simulink model "My_gfm_battery_sil_2_ConvIGBT_zDomain"  (R2025b)
settings: Solver=ode23t  StartTime=0.0  StopTime=10  MaxStep=1e-4  RelTol=1e-3
PreLoadFcn:
  | close all;
  | clear all;
  | clc;
  | 
  | 
  | modelDir = fileparts(get_param(bdroot,'FileName'));
  | 
  | load_system(fullfile(modelDir,'controls_element_lib.slx'));
  | load_system(fullfile(modelDir,'test_sequence_lib.slx'));
  | 
  | Simulink.importExternalCTypes('.\circuitControls_A_autogen.h')
InitFcn:
  | % frequency nominals
  | F_NOM = 60;
  | W_NOM = 2 * pi * F_NOM;
  | 
  | % base values relative to inverter
  | % --------------------------------
  | VLL_INV_NOM = 480;
  | P_INV_NOM = 1e6;
  | Q_INV_NOM = 0.5e6;
  | S_INV_NOM = sqrt(P_INV_NOM^2 + Q_INV_NOM^2);
  | 
  | I_INV_BASE = S_INV_NOM/(sqrt(3)*VLL_INV_NOM);
  | Z_INV_BASE = VLL_INV_NOM^2/S_INV_NOM;
  | L_INV_BASE = Z_INV_BASE / W_NOM;
  | C_INV_BASE = 1 / (Z_INV_BASE * W_NOM);
  | 
  | % nominal ratings for power system model
  | % --------------------------------------
  | INVERTER_COUNT = 100;
  | 
  | VLV_NOM = VLL_INV_NOM;
  | VMV_NOM = 35e3;
  | VHV_NOM = 230e3;
  | S_PLANT = INVERTER_COUNT * S_INV_NOM;
  | 
  | N_GSU = VHV_NOM/VMV_NOM;
  | N_MVT = VMV_NOM/VLV_NOM;
  | 
  | I_LV_BASE = S_PLANT/(sqrt(3)*VLV_NOM);
  | I_MV_BASE = S_PLANT/(sqrt(3)*VMV_NOM);
  | I_HV_BASE = S_PLANT/(sqrt(3)*VHV_NOM);
  | 
  | Z_LV_BASE = VLV_NOM^2/S_PLANT;
  | Z_MV_BASE = VMV_NOM^2/S_PLANT;
  | Z_HV_BASE = VHV_NOM^2/S_PLANT;
  | 
  | L_LV_BASE = Z_LV_BASE / W_NOM;
  | L_MV_BASE = Z_MV_BASE / W_NOM;
  | L_HV_BASE = Z_HV_BASE / W_NOM;
  | C_LV_BASE = 1 / (Z_LV_BASE * W_NOM);
  | C_MV_BASE = 1 / (Z_MV_BASE * W_NOM);
  | C_HV_BASE = 1 / (Z_HV_BASE * W_NOM);
undefined symbols (not defined in the file): D1, D11, Delta, gcbh, j, powergui, SampleTime, sps_rtmsupport, Ts
libraries: simulink x43, spsVoltageMeasurementLib x21, spsThreePhaseSeriesRLCBranchLib x20, spsControlledCurrentSourceLib x20, spsControlledVoltageSourceLib x15, spsThreePhaseVIMeasurementLib x12, spsSeriesRLCBranchLib x11, spsGroundLib x11, test_sequence_lib x10, controls_element_lib x9, spsCurrentMeasurementLib x8, spsThreePhaseTransformerTwoWindingsLib x6
(part 7 of 8)

== system My_gfm_battery_sil_2_ConvIGBT_zDomain/My Inverter Controller /My_machineModel_A/Exciter ==
  note: Aligning with Rotor Frame
      | cos x + j sin x
      | cos (x-120) + j (sin x -120)
      | cos (x+120) + j (sin x +120)
  note: Vb = vd * cos (x-120) - vq * sin (x-120)
  note: Peak EMFa,b,c
  note: Va = vd * cos x - vq * sin x
  note: Vq = 0
  note: Vc = vd * cos (x+120) - vq * sin (x+120)
  Vexc : Inport
  osc[3] : Inport  Port=2
  Constant : Constant  Value=0
  Gain2 : Gain  Gain=1/sqrt(3)
  LPF : Subsystem
  LPF1 : TransferFcn  Commented=on  Denominator=[1/wExciter 1]
  Real-Imag to Complex : RealImagToComplex
  modulator : Subsystem
  v_emf : Outport
  wires:
  LPF/1(Out) -> Gain2/1  "Vref_LL"
  modulator/1(ref) -> v_emf/1
  Gain2/1 -> Real-Imag to Complex/1  "Vref_LN"
  osc[3]/1 -> modulator/2(osc)
  Constant/1 -> Real-Imag to Complex/2
  Real-Imag to Complex/1 -> modulator/1(cmd)
  Vexc/1 -> LPF/1(In)

== system My_gfm_battery_sil_2_ConvIGBT_zDomain/My Inverter Controller /My_machineModel_A/governer ==
  note: Machine enables
  note: RMS LL
  note: RMS LL
  note: Machine Disabled, Power sync on
  Prequest : Inport
  Fref : Inport  Port=2
  enabled : Inport  Port=3
  Vt : Inport  Port=4
  Vq : Inport  Port=5
  f_rotor : Inport  Port=6
  "LPF(DamperDecoupler) limited " : Subsystem
  Saturation1 : Saturate  UpperLimit=nominalFrequency+1  LowerLimit=nominalFrequency-1
  Scope1 : Scope  NumInputPorts=4
      settings: ActiveDisplayYMinimum=-3.88223850701E+6  ActiveDisplayYMaximum=1.39902720117E+6
  Scope2 : Scope  NumInputPorts=3
      settings: ActiveDisplayYMinimum=-4.19262745781E+6  ActiveDisplayYMaximum=4.19262745781E+6  DataLoggingVariableName=ScopeData2
  Sum : Sum  Inputs=|++
  Sum1 : Sum  Inputs=|+-
  Sum2 : Sum  Inputs=++|
  droop power limits : Saturate  UpperLimit=SRated  LowerLimit=-SRated
  k_droop : Gain  Gain=kDroop * SRated
  power request limits : Saturate  UpperLimit=SRated  LowerLimit=-SRated
  synchronizer : Subsystem
  power : Outport
  wires:
  power request limits/1 -> Scope1/1, Sum2/1
  droop power limits/1 -> Sum2/2
  synchronizer/1(p_sync_pu) -> Scope2/1, Sum/2  "p_sync"
  Vq/1 -> synchronizer/1(Vq), Scope2/2
  Prequest/1 -> power request limits/1
  k_droop/1 -> droop power limits/1
  Sum2/1 -> Scope1/2, "LPF(DamperDecoupler) limited "/1(In)
  "LPF(DamperDecoupler) limited "/1(Out) -> Scope1/3, Sum/1  "p_mechanical"
  Saturation1/1 -> Sum1/1
  f_rotor/1 -> Sum1/2
  Fref/1 -> Saturation1/1
  Sum/1 -> Scope1/4, power/1
  Sum1/1 -> k_droop/1
  Vt/1 -> synchronizer/2(Vt), Scope2/3
  enabled/1 -> synchronizer/3(machine_enabled)

== system My_gfm_battery_sil_2_ConvIGBT_zDomain/My Inverter Controller /My_machineModel_A/impedance emulation ==
  v_emf : Inport
  enable : Inport  Port=2
  v_terminal : Inport  Port=3
  Constant : Constant  Value=0
  Integrator : Integrator
  Sum : Sum  Inputs=|+-
  Sum of Elements1 : Sum  Inputs=+
  Sum1 : Sum  Inputs=|+-
  Sum4 : Sum  Inputs=|+-
  Switch : Switch  Criteria=u2 > Threshold  SaturateOnIntegerOverflow=off  InputSameDT=off
  overLs : Gain  Gain=2*pi*60/(Xs * (VllRated^2/SRated))
  rN : Gain  Gain=rn*(VllRated^2/SRated)
  rs : Gain  Gain=rs*(VllRated^2/SRated)
  i_ref : Outport
  wires:
  enable/1 -> Switch/2
  Constant/1 -> Switch/3
  Sum/1 -> Switch/1
  Switch/1 -> Sum4/1
  v_terminal/1 -> Sum/2
  v_emf/1 -> Sum/1
  overLs/1 -> Integrator/1
  Sum of Elements1/1 -> rN/1
  Sum4/1 -> Sum1/1
  Sum1/1 -> overLs/1
  rN/1 -> Sum4/2
  rs/1 -> Sum1/2
  Integrator/1 -> Sum of Elements1/1, rs/1, i_ref/1  "i_ref"

== system My_gfm_battery_sil_2_ConvIGBT_zDomain/My Inverter Controller /My_machineModel_A/power analyzer ==
  iac : Inport
  vac : Inport  Port=2
  Demux1 : Demux  Outputs=3
  Demux2 : Demux  Outputs=3
  Gain3 : Gain  Gain=1 / sqrt(3)
  Product{,1..3} (4 alike) : Product
  Sum of Elements : Sum  Inputs=+
  Sum2 : Sum  Inputs=|+-
  Sum3 : Sum  Inputs=|+-
  Sum4 : Sum  Inputs=|+-
  Sum5 : Sum  Inputs=+++
  P : Outport
  Q : Outport  Port=2
  wires:
  Product/1 -> Sum of Elements/1
  Sum of Elements/1 -> P/1  "P"
  Gain3/1 -> Q/1  "Q"
  Demux1/1 -> Product2/2  "ia"
  Demux2/1 -> Sum2/1, Sum4/2
  Sum2/1 -> Product1/1  "vab"
  Sum5/1 -> Gain3/1
  Sum3/1 -> Product2/1  "vbc"
  iac/1 -> Demux1/1, Product/1
  vac/1 -> Product/2, Demux2/1
  Demux1/2 -> Product3/2  "ib"
  Demux1/3 -> Product1/2  "ic"
  Demux2/3 -> Sum3/2, Sum4/1
  Demux2/2 -> Sum2/2, Sum3/1
  Product3/1 -> Sum5/2
  Sum4/1 -> Product3/1  "vca"
  Product2/1 -> Sum5/3
  Product1/1 -> Sum5/1

== system My_gfm_battery_sil_2_ConvIGBT_zDomain/My Inverter Controller /My_machineModel_A/rotor model ==
  p_mechanical : Inport
  p_electrical : Inport  Port=2
  Constant : Constant  Value=nominalFrequency
  HPF (wDamperDecoupler) : TransferFcn  Commented=on  Numerator=[0.3 0]  Denominator=[0.3 1]
  HPF (wDamperDecoupler) 1 : Subsystem
  Integrator1 : Integrator  LimitOutput=on  UpperSaturationLimit=5  LowerSaturationLimit=-5
  Sum : Sum  Inputs=++|
  Sum2 : Sum  Inputs=|+-
  Sum3 : Sum  Inputs=|+-
  k_damp : Gain  Gain=kDamper*SRated
  k_inertia : Gain  Gain=(nominalFrequency/2)/(inertialConstant*SRated)
  oscillator_3ph : Subsystem
  osc[3] : Outport
  f_rotor : Outport  Port=2
  wires:
  Constant/1 -> Sum/1
  Sum/1 -> oscillator_3ph/1(f), f_rotor/1
  k_damp/1 -> Sum2/2
  Integrator1/1 -> HPF (wDamperDecoupler) 1/1(in), Sum/2
  p_mechanical/1 -> Sum3/1
  Sum3/1 -> Sum2/1
  p_electrical/1 -> Sum3/2
  HPF (wDamperDecoupler) 1/1(out) -> k_damp/1
  oscillator_3ph/1(osc[3]) -> osc[3]/1
  k_inertia/1 -> Integrator1/1
  Sum2/1 -> k_inertia/1

== system My_gfm_battery_sil_2_ConvIGBT_zDomain/My Inverter Controller /My_machineModel_A/voltage analyzer ==
  osc[3] : Inport
  v_terminal : Inport  Port=2
  Complex to Magnitude-Angle : ComplexToMagnitudeAngle
  Complex to Real-Imag : ComplexToRealImag
  Conj : Math  Operator=conj  SignedPower=on
  LPF : Subsystem
  "LPF " : Subsystem
  Product1 : Product
  Product2 : Product
  Real-Imag to Complex1 : RealImagToComplex
  Sum of Elements1 : Sum  Inputs=+
  Sum of Elements2 : Sum  Inputs=+
  Terminator : Terminator
  over_sqrt(3) : Gain  Gain=1/sqrt(3)
  over_sqrt(3)1 : Gain  Gain=1/sqrt(3)
  sqrt(2) : Gain  Gain=sqrt(2)
  Vd : Outport
  Vq : Outport  Port=2
  Vt_Mag : Outport  Port=3
  wires:
  "LPF "/1(Out) -> Real-Imag to Complex1/2, Vq/1  "Vq"
  osc[3]/1 -> Conj/1
  LPF/1(Out) -> Real-Imag to Complex1/1, Vd/1  "Vd"
  over_sqrt(3)1/1 -> LPF/1(In)
  over_sqrt(3)/1 -> "LPF "/1(In)
  Complex to Real-Imag/1 -> Product2/1
  Complex to Real-Imag/2 -> Product1/1
  Sum of Elements2/1 -> over_sqrt(3)1/1
  v_terminal/1 -> Product2/2, Product1/2
  Product1/1 -> Sum of Elements1/1
  Sum of Elements1/1 -> over_sqrt(3)/1
  sqrt(2)/1 -> Complex to Real-Imag/1
  Conj/1 -> sqrt(2)/1
  Product2/1 -> Sum of Elements2/1
  Complex to Magnitude-Angle/1 -> Vt_Mag/1  "Vt"
  Real-Imag to Complex1/1 -> Complex to Magnitude-Angle/1  "Vd"
  Complex to Magnitude-Angle/2 -> Terminator/1

== system My_gfm_battery_sil_2_ConvIGBT_zDomain/My Inverter Controller /My_machineModel_A1/excitation ==
  note: This limit is needed to avoid excessive currents during blackstart that cause windup in current limiting logic.. It results in a linear ramp of voltage during blackstart
  note: Using asym filter to traget long extended low voltage events, prevent it from acting during typical faults
  note: Aligning with Rotor Frame
      | cos x + j sin x
      | cos (x-120) + j (sin x -120)
      | cos (x+120) + j (sin x +120)
  note: Vb = vd * cos (x-120) - vq * sin (x-120)
  note: Peak EMFa,b,c
  note: Va = vd * cos x - vq * sin x
  note: Vq = 0
  note: Vc = vd * cos (x+120) - vq * sin (x+120)
  VRef : Inport
  osc[3] : Inport  Port=2
  Vt : Inport  Port=3
  Constant : Constant  Value=0
  Gain2 : Gain  Gain=1/sqrt(3)
  LPF : Subsystem
  LPF1 : TransferFcn  Commented=on  Denominator=[1/wExciter 1]
  Min : MinMax  Inputs=2
  Real-Imag to Complex : RealImagToComplex
  Saturation1 : Saturate  UpperLimit=1.1*VllRated  LowerLimit=0.9*VllRated
  Sum : Sum  Inputs=++|
  assymmetric filter1 : Subsystem
  modulator : Subsystem
  voltage_headroom : Constant  Value=0.3*VllRated
  v_emf : Outport
  wires:
  Sum/1 -> Min/2
  Saturation1/1 -> Min/1
  voltage_headroom/1 -> Sum/1
  LPF/1(Out) -> Gain2/1  "Vref_LL"
  Min/1 -> LPF/1(In)
  VRef/1 -> Saturation1/1  "VRef"
  modulator/1(ref) -> v_emf/1
  assymmetric filter1/1(out) -> Sum/2  "Vt_conditioned"
  Vt/1 -> assymmetric filter1/1(in)  "Vt"
  Gain2/1 -> Real-Imag to Complex/1  "Vref_LN"
  osc[3]/1 -> modulator/2(osc)
  Constant/1 -> Real-Imag to Complex/2
  Real-Imag to Complex/1 -> modulator/1(cmd)

== system My_gfm_battery_sil_2_ConvIGBT_zDomain/My Inverter Controller /My_machineModel_A1/governer ==
  note: Machine enables
  note: RMS LL
  note: RMS LL
  note: Machine Disabled, Power sync on
  Prequest : Inport
  Fref : Inport  Port=2
  enabled : Inport  Port=3
  Vt : Inport  Port=4
  Vq : Inport  Port=5
  f_rotor : Inport  Port=6
  "LPF(DamperDecoupler) limited " : Subsystem
  Saturation1 : Saturate  UpperLimit=nominalFrequency+1  LowerLimit=nominalFrequency-1
  Scope1 : Scope  NumInputPorts=4
      settings: ActiveDisplayYMinimum=-3.88223850701E+6  ActiveDisplayYMaximum=1.39902720117E+6
  Scope2 : Scope  NumInputPorts=3
      settings: ActiveDisplayYMinimum=-4.19262745781E+6  ActiveDisplayYMaximum=4.19262745781E+6  DataLoggingVariableName=ScopeData2
  Sum : Sum  Inputs=|++
  Sum1 : Sum  Inputs=|+-
  Sum2 : Sum  Inputs=++|
  droop power limits : Saturate  UpperLimit=SRated  LowerLimit=-SRated
  k_droop : Gain  Gain=kDroop * SRated
  power request limits : Saturate  UpperLimit=SRated  LowerLimit=-SRated
  synchronizer : Subsystem
  power : Outport
  wires:
  power request limits/1 -> Scope1/1, Sum2/1
  droop power limits/1 -> Sum2/2
  synchronizer/1(p_sync_pu) -> Scope2/1, Sum/2  "p_sync"
  Vq/1 -> Scope2/2, synchronizer/1(Vq)
  Prequest/1 -> power request limits/1
  k_droop/1 -> droop power limits/1
  Sum2/1 -> Scope1/2, "LPF(DamperDecoupler) limited "/1(In)
  "LPF(DamperDecoupler) limited "/1(Out) -> Scope1/3, Sum/1  "p_mechanical"
  Saturation1/1 -> Sum1/1
  f_rotor/1 -> Sum1/2
  Fref/1 -> Saturation1/1
  Sum/1 -> Scope1/4, power/1
  Sum1/1 -> k_droop/1
  Vt/1 -> Scope2/3, synchronizer/2(Vt)
  enabled/1 -> synchronizer/3(machine_enabled)

== system My_gfm_battery_sil_2_ConvIGBT_zDomain/My Inverter Controller /My_machineModel_A1/governer1 ==
  note: Machine enables
  note: RMS LL
  note: RMS LL
  note: Machine Disabled, Power sync on
  Prequest : Inport
  Fref : Inport  Port=2
  enabled : Inport  Port=3
  Vd : Inport  Port=4
  Vq : Inport  Port=5
  f_rotor : Inport  Port=6
  LPF(DamperDecoupler) - limited : Subsystem  Commented=on
  LPF(DamperDecoupler) limited 1 : Subsystem
  Saturation1 : Saturate  UpperLimit=nominalFrequency+1  LowerLimit=nominalFrequency-1
  Sum : Sum  Inputs=|++
  Sum1 : Sum  Inputs=|+-
  Sum2 : Sum  Inputs=++|
  droop power limits : Saturate  UpperLimit=SRated  LowerLimit=-SRated
  k_droop : Gain  Gain=kDroop * SRated
  power request limits : Saturate  UpperLimit=SRated  LowerLimit=-SRated
  synchronizer : Subsystem
  power : Outport
  wires:
  power request limits/1 -> Sum2/1
  droop power limits/1 -> Sum2/2
  synchronizer/1(p_sync_pu) -> Sum/2  "p_sync"
  Vq/1 -> synchronizer/1(Vq)
  Prequest/1 -> power request limits/1
  k_droop/1 -> droop power limits/1
  Sum2/1 -> LPF(DamperDecoupler) limited 1/1(In)
  enabled/1 -> synchronizer/3(machine_enabled)
  LPF(DamperDecoupler) limited 1/1(Out) -> Sum/1  "p_mechanical"
  Saturation1/1 -> Sum1/1
  f_rotor/1 -> Sum1/2
  Fref/1 -> Saturation1/1
  Sum/1 -> power/1
  Sum1/1 -> k_droop/1
  Vd/1 -> synchronizer/2(Vd)

== system My_gfm_battery_sil_2_ConvIGBT_zDomain/My Inverter Controller /My_machineModel_A1/impedance emulation ==
  v_emf : Inport
  enable : Inport  Port=2
  v_terminal : Inport  Port=3
  Constant : Constant  Value=0
  Integrator : Integrator
  Sum : Sum  Inputs=|+-
  Sum of Elements1 : Sum  Inputs=+
  Sum1 : Sum  Inputs=|+-
  Sum4 : Sum  Inputs=|+-
  Switch : Switch  Criteria=u2 > Threshold  SaturateOnIntegerOverflow=off  InputSameDT=off
  overLs : Gain  Gain=2*pi*60/(Xs * (VllRated^2/SRated))
  rN : Gain  Gain=0.2*(VllRated^2/SRated)
  rs : Gain  Gain=rs*(VllRated^2/SRated)
  i_ref : Outport
  wires:
  enable/1 -> Switch/2
  Constant/1 -> Switch/3
  Sum/1 -> Switch/1
  Switch/1 -> Sum4/1
  v_terminal/1 -> Sum/2
  v_emf/1 -> Sum/1
  overLs/1 -> Integrator/1
  Sum of Elements1/1 -> rN/1
  Sum4/1 -> Sum1/1
  Sum1/1 -> overLs/1
  rN/1 -> Sum4/2
  rs/1 -> Sum1/2
  Integrator/1 -> Sum of Elements1/1, rs/1, i_ref/1  "i_ref"

== system My_gfm_battery_sil_2_ConvIGBT_zDomain/My Inverter Controller /My_machineModel_A1/power analyzer ==
  iac : Inport
  vac : Inport  Port=2
  Demux1 : Demux  Outputs=3
  Demux2 : Demux  Outputs=3
  Gain3 : Gain  Gain=1 / sqrt(3)
  Product{,1..3} (4 alike) : Product
  Sum of Elements : Sum  Inputs=+
  Sum2 : Sum  Inputs=|+-
  Sum3 : Sum  Inputs=|+-
  Sum4 : Sum  Inputs=|+-
  Sum5 : Sum  Inputs=+++
  P : Outport
  Q : Outport  Port=2
  wires:
  Product/1 -> Sum of Elements/1
  Sum of Elements/1 -> P/1  "P"
  Gain3/1 -> Q/1  "Q"
  Demux1/1 -> Product2/2  "ia"
  Demux2/1 -> Sum2/1, Sum4/2
  Sum2/1 -> Product1/1  "vab"
  Sum5/1 -> Gain3/1
  Sum3/1 -> Product2/1  "vbc"
  iac/1 -> Demux1/1, Product/1
  vac/1 -> Product/2, Demux2/1
  Demux1/2 -> Product3/2  "ib"
  Demux1/3 -> Product1/2  "ic"
  Demux2/3 -> Sum3/2, Sum4/1
  Demux2/2 -> Sum2/2, Sum3/1
  Product3/1 -> Sum5/2
  Sum4/1 -> Product3/1  "vca"
  Product2/1 -> Sum5/3
  Product1/1 -> Sum5/1

== system My_gfm_battery_sil_2_ConvIGBT_zDomain/My Inverter Controller /My_machineModel_A1/rotor model ==
  p_mechanical : Inport
  p_electrical : Inport  Port=2
  Constant : Constant  Value=nominalFrequency
  HPF (wDamperDecoupler) : TransferFcn  Commented=on  Numerator=[0.3 0]  Denominator=[0.3 1]
  HPF (wDamperDecoupler) 1 : Subsystem
  Integrator1 : Integrator  LimitOutput=on  UpperSaturationLimit=5  LowerSaturationLimit=-5
  Sum : Sum  Inputs=++|
  Sum2 : Sum  Inputs=|+-
  Sum3 : Sum  Inputs=|+-
  k_damp : Gain  Gain=kDamper*SRated
  k_inertia : Gain  Gain=(nominalFrequency/2)/(inertialConstant*SRated)
  oscillator_3ph : Subsystem
  osc[3] : Outport
  f_rotor : Outport  Port=2
  wires:
  Constant/1 -> Sum/1
  Sum/1 -> oscillator_3ph/1(f), f_rotor/1
  k_damp/1 -> Sum2/2
  Integrator1/1 -> HPF (wDamperDecoupler) 1/1(in), Sum/2
  p_mechanical/1 -> Sum3/1
  Sum3/1 -> Sum2/1
  p_electrical/1 -> Sum3/2
  HPF (wDamperDecoupler) 1/1(out) -> k_damp/1
  oscillator_3ph/1(osc[3]) -> osc[3]/1
  k_inertia/1 -> Integrator1/1
  Sum2/1 -> k_inertia/1

== system My_gfm_battery_sil_2_ConvIGBT_zDomain/My Inverter Controller /My_machineModel_A1/voltage analyzer ==
  osc[3] : Inport
  v_terminal : Inport  Port=2
  Complex to Magnitude-Angle : ComplexToMagnitudeAngle
  Complex to Real-Imag : ComplexToRealImag
  Conj : Math  Operator=conj  SignedPower=on
  Product1 : Product
  Product2 : Product
  Real-Imag to Complex1 : RealImagToComplex
  Sum of Elements1 : Sum  Inputs=+
  Sum of Elements2 : Sum  Inputs=+
  Terminator : Terminator
  Transfer Fcn : TransferFcn  Denominator=[0.02 1]
  Transfer Fcn1 : TransferFcn  Denominator=[0.02 1]
  over_sqrt(3) : Gain  Gain=1/sqrt(3)
  over_sqrt(3)1 : Gain  Gain=1/sqrt(3)
  sqrt(2) : Gain  Gain=sqrt(2)
  Vd : Outport
  Vq : Outport  Port=2
  Vt_Mag : Outport  Port=3
  wires:
  Transfer Fcn/1 -> Real-Imag to Complex1/2, Vq/1  "Vq"
  osc[3]/1 -> Conj/1
  Transfer Fcn1/1 -> Real-Imag to Complex1/1, Vd/1  "Vd"
  over_sqrt(3)1/1 -> Transfer Fcn1/1
  over_sqrt(3)/1 -> Transfer Fcn/1
  Complex to Real-Imag/1 -> Product2/1
  Complex to Real-Imag/2 -> Product1/1
  Sum of Elements2/1 -> over_sqrt(3)1/1
  v_terminal/1 -> Product2/2, Product1/2
  Product1/1 -> Sum of Elements1/1
  Sum of Elements1/1 -> over_sqrt(3)/1
  sqrt(2)/1 -> Complex to Real-Imag/1
  Conj/1 -> sqrt(2)/1
  Product2/1 -> Sum of Elements2/1
  Complex to Magnitude-Angle/1 -> Vt_Mag/1  "Vt"
  Real-Imag to Complex1/1 -> Complex to Magnitude-Angle/1  "Vd"
  Complex to Magnitude-Angle/2 -> Terminator/1

== system My_gfm_battery_sil_2_ConvIGBT_zDomain/Plant controller (simplified example)/LVRT_foldback/LPF ==
  in : Inport
  1/0.01 : Gain  Gain=1/0.01
  Integrator : Integrator
  Sum3 : Sum  Inputs=|+-
  out : Outport
  wires:
  Integrator/1 -> out/1, Sum3/2
  Sum3/1 -> 1/0.01/1
  in/1 -> Sum3/1
  1/0.01/1 -> Integrator/1

== system My_gfm_battery_sil_2_ConvIGBT_zDomain/Plant controller (simplified example)/LVRT_foldback/assymmetric filter ==
  in : Inport
  Gain1 : Gain  Gain=1/0.01
  Integrator : Integrator
  Saturation1 : Saturate  UpperLimit=0.05 * 1  LowerLimit=-1 * 1
  Sum3 : Sum  Inputs=|+-
  out : Outport
  wires:
  Integrator/1 -> out/1, Sum3/2
  Sum3/1 -> Saturation1/1
  in/1 -> Sum3/1
  Gain1/1 -> Integrator/1
  Saturation1/1 -> Gain1/1

== system My_gfm_battery_sil_2_ConvIGBT_zDomain/Plant controller (simplified example)/Meter/PLL-analog ==
  note: cos x - j sin x
      | cos (x-120) - j (sin x -120)
      | cos (x+120) - j (sin x +120)
  note: cos x + j sin x
      | cos (x-120) + j (sin x -120)
      | cos (x+120) + j (sin x +120)
  note: -sin x
      |  -sin (x -120)
      |  -sin (x +120)
  note: cos x + j sin x
      | cos (x-120) + j (sin x -120)
      | cos (x+120) + j (sin x +120)
  ref : Inport
  Complex to Real-Imag : ComplexToRealImag
  Conj : Math  Operator=conj  SignedPower=on
  Gain : Gain  Gain=3
  Gain2 : Gain  Gain=30
  Integrator : Integrator  LimitOutput=on  UpperSaturationLimit=5  LowerSaturationLimit=-5
  Product2 : Product
  Saturation : Saturate  UpperLimit=5  LowerLimit=-5
  Sum of Elements : Sum  Inputs=+
  Sum1 : Sum  Inputs=|++
  Sum2 : Sum  Inputs=|++
  Terminator : Terminator
  Transfer Fcn : TransferFcn  Denominator=[0.02 1]
  fnom : Constant  Value=60
  oscillator_3ph : Subsystem
  freq : Outport
  osc : Outport  Port=2
  wires:
  Gain2/1 -> Integrator/1
  Integrator/1 -> Sum2/2
  Sum2/1 -> Sum1/1
  fnom/1 -> Sum1/2
  Product2/1 -> Sum of Elements/1
  Transfer Fcn/1 -> Gain/1, Gain2/1
  Saturation/1 -> Sum2/1
  Gain/1 -> Saturation/1
  Sum1/1 -> oscillator_3ph/1(f), freq/1
  ref/1 -> Product2/1
  Sum of Elements/1 -> Transfer Fcn/1
  Conj/1 -> Complex to Real-Imag/1
  Complex to Real-Imag/1 -> Terminator/1
  Complex to Real-Imag/2 -> Product2/2
  oscillator_3ph/1(osc[3]) -> osc/1, Conj/1

== system My_gfm_battery_sil_2_ConvIGBT_zDomain/Plant controller (simplified example)/VoltVAr/LPF ==
  in : Inport
  1/0.05 : Gain  Gain=1/0.05
  Integrator : Integrator
  Sum3 : Sum  Inputs=|+-
  out : Outport
  wires:
  Integrator/1 -> out/1, Sum3/2
  Sum3/1 -> 1/0.05/1
  in/1 -> Sum3/1
  1/0.05/1 -> Integrator/1

== system My_gfm_battery_sil_2_ConvIGBT_zDomain/Plant controller (simplified example)/VoltVAr/LPF1 ==
  in : Inport
  1/0.05 : Gain  Gain=1/0.05
  1/0.1 : Gain
  Integrator : Integrator
  Saturation : Saturate  UpperLimit=inf  LowerLimit=0
  Saturation1 : Saturate  UpperLimit=0  LowerLimit=-inf
  Sum : Sum  Inputs=|++
  Sum3 : Sum  Inputs=|+-
  out : Outport
  wires:
  Integrator/1 -> out/1, Sum3/2
  Sum3/1 -> 1/0.1/1, 1/0.05/1
  in/1 -> Sum3/1
  1/0.05/1 -> Saturation/1
  Sum/1 -> Integrator/1
  1/0.1/1 -> Saturation1/1
  Saturation/1 -> Sum/1
  Saturation1/1 -> Sum/2

== system My_gfm_battery_sil_2_ConvIGBT_zDomain/ac Network with MVT (native math)3/Two-Level Converter/Model1 ==
  note: (Uref)
  g : Inport  SampleTime=Ts
  Block : Inport  Port=2
  Add : Sum  Inputs=+-
  Constant : Constant
  Constant1 : Constant  Value=0
  Constant2 : Constant
  Current Measurement : spsCurrentMeasurementLib/Current Measurement  PhasorSimulation=off  OutputType=Complex  PSBequivalent=0
  Data Type Conversion2 : DataTypeConversion  OutDataTypeStr=double  SaturateOnIntegerOverflow=off  RndMeth=Floor
  Demux : Demux  Outputs=2
  Fcn2 : Fcn  Expr=(u(1)+1)*0.5
  MATLAB Function : MATLAB Function  TreatAsAtomicUnit=on
  Mux : Mux  Inputs=2
  Mux1 : Mux  Inputs=2
  Power : spsHalfBridgeModel/Power  SystemSampleTime=-1  VariantActivationTime=update diagram  EmptyChoice=off  PassThrough=off  PassThroughVariantControl=(default)  EmptyChoiceVariantControl=(default)  AllowFlexibleInterface=on  Latency=0  AutoFrameSizeCalculation=off
  Product2 : Product
  Product8 : Product
  Saturation : Saturate  UpperLimit=1.0  LowerLimit=-1.0
  Scope : Scope  NumInputPorts=2
      settings: ActiveDisplayYMinimum=-0.125  ActiveDisplayYMaximum=1.125
  Scope1 : Scope  NumInputPorts=2
      settings: ActiveDisplayYMinimum=0.0581  ActiveDisplayYMaximum=0.93277  DataLoggingVariableName=ScopeData2
  Scope2 : Scope  NumInputPorts=6
      settings: ActiveDisplayYMinimum=-1057.03298  ActiveDisplayYMaximum=1237.20421  DataLoggingVariableName=ScopeData3
  Switch : Switch  Criteria=u2 > Threshold  SaturateOnIntegerOverflow=off  InputSameDT=off
  Transfer Fcn : TransferFcn  Denominator=[1e-6 1]
  Transfer Fcn1 : TransferFcn  Denominator=[1e-6 1]
  Transfer Fcn2 : TransferFcn  Denominator=[1e-6 1]
  Voltage Measurement : spsVoltageMeasurementLib/Voltage Measurement  PhasorSimulation=off  OutputType=Complex  PSBequivalent=0
  + : PMIOPort  Tag=PMCPort  Side=Right
  - : PMIOPort  Tag=PMCPort  Port=2  Side=Right
  Out : PMIOPort  Tag=PMCPort  Port=3  Side=Left
  wires:
  Saturation/1 -> Fcn2/1
  g/1 -> Saturation/1
  Block/1 -> Switch/2, Scope/1
  Data Type Conversion2/1 -> Scope/2, Product2/1, Product8/1
  Product2/1 -> Mux1/1
  Product8/1 -> Mux1/2
  Add/1 -> Scope1/2, Product8/2
  Constant/1 -> Add/1
  Fcn2/1 -> Add/2, Scope1/1, Product2/2
  Switch/1 -> Data Type Conversion2/1
  Power/2 -> Scope2/4, Demux/1
  Demux/2 -> Transfer Fcn2/1
  Demux/1 -> Transfer Fcn/1
  Transfer Fcn/1 -> Mux/1
  Transfer Fcn2/1 -> Mux/2
  Mux/1 -> MATLAB Function/3(I)
  Transfer Fcn1/1 -> MATLAB Function/2(Vdc)
  Power/1 -> Scope2/2, Transfer Fcn1/1
  MATLAB Function/2(Idc) -> Power/2, Scope2/3
  MATLAB Function/1(V) -> Power/1, Scope2/1
  Mux1/1 -> MATLAB Function/1(g)
  Constant1/1 -> Switch/1
  Constant2/1 -> Switch/3
  Voltage Measurement/1 -> Scope2/5
  Current Measurement/1 -> Scope2/6
  connections:
  Power/LConn1 -- Current Measurement/LConn1 -- Voltage Measurement/LConn1
  Power/RConn2 -- Voltage Measurement/LConn2 -- -/RConn1
  Power/RConn1 -- +/RConn1
  Current Measurement/RConn1 -- Out/RConn1

== system My_gfm_battery_sil_2_ConvIGBT_zDomain/ac Network with MVT (native math)3/Two-Level Converter/Model2 ==
  note: (Uref)
  g : Inport  SampleTime=Ts
  Block : Inport  Port=2
  Add : Sum  Inputs=+-
  Constant : Constant
  Constant1 : Constant  Value=0
  Constant2 : Constant
  Data Type Conversion2 : DataTypeConversion  OutDataTypeStr=double  SaturateOnIntegerOverflow=off  RndMeth=Floor
  Demux : Demux  Outputs=2
  Fcn2 : Fcn  Expr=(u(1)+1)*0.5
  MATLAB Function : MATLAB Function  TreatAsAtomicUnit=on
  Mux : Mux  Inputs=2
  Mux1 : Mux  Inputs=2
  Power : spsHalfBridgeModel/Power  SystemSampleTime=-1  VariantActivationTime=update diagram  EmptyChoice=off  PassThrough=off  PassThroughVariantControl=(default)  EmptyChoiceVariantControl=(default)  AllowFlexibleInterface=on  Latency=0  AutoFrameSizeCalculation=off
  Product2 : Product
  Product8 : Product
  Saturation : Saturate  UpperLimit=1.0  LowerLimit=-1.0
  Scope : Scope  NumInputPorts=2
      settings: ActiveDisplayYMinimum=-0.125  ActiveDisplayYMaximum=1.125
  Scope1 : Scope  NumInputPorts=2
      settings: ActiveDisplayYMinimum=-0.0256  ActiveDisplayYMaximum=0.96024  DataLoggingVariableName=ScopeData2
  Scope2 : Scope  NumInputPorts=5
      settings: ActiveDisplayYMinimum=-1250  ActiveDisplayYMaximum=1079.00943  DataLoggingVariableName=ScopeData3
  Switch : Switch  Criteria=u2 > Threshold  SaturateOnIntegerOverflow=off  InputSameDT=off
  Transfer Fcn : TransferFcn  Denominator=[1e-6 1]
  Transfer Fcn1 : TransferFcn  Denominator=[1e-6 1]
  Transfer Fcn2 : TransferFcn  Denominator=[1e-6 1]
  Voltage Measurement : spsVoltageMeasurementLib/Voltage Measurement  PhasorSimulation=off  OutputType=Complex  PSBequivalent=0
  + : PMIOPort  Tag=PMCPort  Side=Right
  - : PMIOPort  Tag=PMCPort  Port=2  Side=Right
  Out : PMIOPort  Tag=PMCPort  Port=3  Side=Left
  wires:
  Saturation/1 -> Fcn2/1
  g/1 -> Saturation/1
  Block/1 -> Switch/2, Scope/1
  Data Type Conversion2/1 -> Scope/2, Product2/1, Product8/1
  Product2/1 -> Mux1/1
  Product8/1 -> Mux1/2
  Add/1 -> Scope1/2, Product8/2
  Constant/1 -> Add/1
  Fcn2/1 -> Add/2, Scope1/1, Product2/2
  Switch/1 -> Data Type Conversion2/1
  Power/2 -> Scope2/4, Demux/1
  Demux/2 -> Transfer Fcn2/1
  Demux/1 -> Transfer Fcn/1
  Transfer Fcn/1 -> Mux/1
  Transfer Fcn2/1 -> Mux/2
  Mux/1 -> MATLAB Function/3(I)
  Transfer Fcn1/1 -> MATLAB Function/2(Vdc)
  Power/1 -> Scope2/2, Transfer Fcn1/1
  MATLAB Function/2(Idc) -> Power/2, Scope2/3
  MATLAB Function/1(V) -> Power/1, Scope2/1
  Mux1/1 -> MATLAB Function/1(g)
  Constant1/1 -> Switch/1
  Constant2/1 -> Switch/3
  Voltage Measurement/1 -> Scope2/5
  connections:
  Out/RConn1 -- Power/LConn1 -- Voltage Measurement/LConn1
  -/RConn1 -- Power/RConn2 -- Voltage Measurement/LConn2
  Power/RConn1 -- +/RConn1

== system My_gfm_battery_sil_2_ConvIGBT_zDomain/ac Network with MVT (native math)3/Two-Level Converter/Model3 ==
  note: (Uref)
  g : Inport  SampleTime=Ts
  Block : Inport  Port=2
  Add : Sum  Inputs=+-
  Constant : Constant
  Constant1 : Constant  Value=0
  Constant2 : Constant
  Data Type Conversion2 : DataTypeConversion  OutDataTypeStr=double  SaturateOnIntegerOverflow=off  RndMeth=Floor
  Demux : Demux  Outputs=2
  Fcn2 : Fcn  Expr=(u(1)+1)*0.5
  MATLAB Function : MATLAB Function  TreatAsAtomicUnit=on
  Mux : Mux  Inputs=2
  Mux1 : Mux  Inputs=2
  Power : spsHalfBridgeModel/Power  SystemSampleTime=-1  VariantActivationTime=update diagram  EmptyChoice=off  PassThrough=off  PassThroughVariantControl=(default)  EmptyChoiceVariantControl=(default)  AllowFlexibleInterface=on  Latency=0  AutoFrameSizeCalculation=off
  Product2 : Product
  Product8 : Product
  Saturation : Saturate  UpperLimit=1.0  LowerLimit=-1.0
  Scope : Scope  NumInputPorts=2
      settings: ActiveDisplayYMinimum=-0.125  ActiveDisplayYMaximum=1.125
  Scope1 : Scope  NumInputPorts=2
      settings: ActiveDisplayYMinimum=-0.0256  ActiveDisplayYMaximum=0.96024  DataLoggingVariableName=ScopeData2
  Scope2 : Scope  NumInputPorts=5
      settings: ActiveDisplayYMinimum=-1250  ActiveDisplayYMaximum=1079.00943  DataLoggingVariableName=ScopeData3
  Switch : Switch  Criteria=u2 > Threshold  SaturateOnIntegerOverflow=off  InputSameDT=off
  Transfer Fcn : TransferFcn  Denominator=[1e-6 1]
  Transfer Fcn1 : TransferFcn  Denominator=[1e-6 1]
  Transfer Fcn2 : TransferFcn  Denominator=[1e-6 1]
  Voltage Measurement : spsVoltageMeasurementLib/Voltage Measurement  PhasorSimulation=off  OutputType=Complex  PSBequivalent=0
  + : PMIOPort  Tag=PMCPort  Side=Right
  - : PMIOPort  Tag=PMCPort  Port=2  Side=Right
  Out : PMIOPort  Tag=PMCPort  Port=3  Side=Left
  wires:
  Saturation/1 -> Fcn2/1
  g/1 -> Saturation/1
  Block/1 -> Switch/2, Scope/1
  Data Type Conversion2/1 -> Scope/2, Product2/1, Product8/1
  Product2/1 -> Mux1/1
  Product8/1 -> Mux1/2
  Add/1 -> Scope1/2, Product8/2
  Constant/1 -> Add/1
  Fcn2/1 -> Add/2, Scope1/1, Product2/2
  Switch/1 -> Data Type Conversion2/1
  Power/2 -> Scope2/4, Demux/1
  Demux/2 -> Transfer Fcn2/1
  Demux/1 -> Transfer Fcn/1
  Transfer Fcn/1 -> Mux/1
  Transfer Fcn2/1 -> Mux/2
  Mux/1 -> MATLAB Function/3(I)
  Transfer Fcn1/1 -> MATLAB Function/2(Vdc)
  Power/1 -> Scope2/2, Transfer Fcn1/1
  MATLAB Function/2(Idc) -> Power/2, Scope2/3
  MATLAB Function/1(V) -> Power/1, Scope2/1
  Mux1/1 -> MATLAB Function/1(g)
  Constant1/1 -> Switch/1
  Constant2/1 -> Switch/3
  Voltage Measurement/1 -> Scope2/5
  connections:
  Out/RConn1 -- Power/LConn1 -- Voltage Measurement/LConn1
  -/RConn1 -- Power/RConn2 -- Voltage Measurement/LConn2
  Power/RConn1 -- +/RConn1

== system My_gfm_battery_sil_2_ConvIGBT_zDomain/ac Network with MVT (native math)4/Network Interface/CSI2 ==
  I : Inport
  Demux : Demux  Outputs=3
  Series RLC Branch : spsSeriesRLCBranchLib/Series RLC Branch  LConnTagsString=__new0  RConnTagsString=__new0  BranchType=R  Resistance=1e3  Inductance=1e-3  SetiL0=off  InitialCurrent=0  Capacitance=1e-6  Setx0=off  InitialVoltage=0  Measurements=None
  Series RLC Branch1 : spsSeriesRLCBranchLib/Series RLC Branch  LConnTagsString=__new0  RConnTagsString=__new0  BranchType=R  Resistance=1e3  Inductance=1e-3  SetiL0=off  InitialCurrent=0  Capacitance=1e-6  Setx0=off  InitialVoltage=0  Measurements=None
  Series RLC Branch2 : spsSeriesRLCBranchLib/Series RLC Branch  LConnTagsString=__new0  RConnTagsString=__new0  BranchType=R  Resistance=1e3  Inductance=1e-3  SetiL0=off  InitialCurrent=0  Capacitance=1e-6  Setx0=off  InitialVoltage=0  Measurements=None
  iA : spsControlledCurrentSourceLib/Controlled Current Source  Initialize=off  Source_Type=AC  Amplitude=0  Phase=0  Frequency=0  Measurements=None
  iB : spsControlledCurrentSourceLib/Controlled Current Source  Initialize=off  Source_Type=AC  Amplitude=0  Phase=0  Frequency=0  Measurements=None
  iB1 : spsControlledCurrentSourceLib/Controlled Current Source  Initialize=off  Source_Type=AC  Amplitude=0  Phase=0  Frequency=0  Measurements=None
  A : PMIOPort  Side=Right
  B : PMIOPort  Port=2  Side=Right
  C : PMIOPort  Port=3  Side=Right
  wires:
  Demux/1 -> iA/1
  Demux/2 -> iB/1
  I/1 -> Demux/1
  Demux/3 -> iB1/1
  connections:
  iA/RConn1 -- A/RConn1 -- Series RLC Branch/LConn1
  iB/RConn1 -- B/RConn1 -- Series RLC Branch1/LConn1
  Series RLC Branch1/RConn1 -- Series RLC Branch/RConn1 -- iA/LConn1 -- iB/LConn1 -- iB1/LConn1 -- Series RLC Branch2/RConn1
  C/RConn1 -- iB1/RConn1 -- Series RLC Branch2/LConn1

== system My_gfm_battery_sil_2_ConvIGBT_zDomain/ac Network with MVT (native math)4/Network Interface/Cur Meas ==
  Current Measurement : spsCurrentMeasurementLib/Current Measurement  PhasorSimulation=off  OutputType=Complex  PSBequivalent=0
  Current Measurement1 : spsCurrentMeasurementLib/Current Measurement  PhasorSimulation=off  OutputType=Complex  PSBequivalent=0
  Current Measurement2 : spsCurrentMeasurementLib/Current Measurement  PhasorSimulation=off  OutputType=Complex  PSBequivalent=0
  Mux : Mux  Inputs=3
  A : PMIOPort  Side=Left
  B : PMIOPort  Port=2  Side=Left
  C : PMIOPort  Port=3  Side=Left
  a : PMIOPort  Port=4  Side=Right
  b : PMIOPort  Port=5  Side=Right
  c : PMIOPort  Port=6  Side=Right
  I : Outport  VectorParamsAs1DForOutWhenUnconnected=off
  wires:
  Current Measurement/1 -> Mux/1
  Current Measurement1/1 -> Mux/2
  Mux/1 -> I/1
  Current Measurement2/1 -> Mux/3
  connections:
  Current Measurement1/LConn1 -- B/RConn1
  Current Measurement/LConn1 -- A/RConn1
  Current Measurement2/LConn1 -- C/RConn1
  a/RConn1 -- Current Measurement/RConn1
  b/RConn1 -- Current Measurement1/RConn1
  c/RConn1 -- Current Measurement2/RConn1

== system My_gfm_battery_sil_2_ConvIGBT_zDomain/ac Network with MVT (native math)4/Network Interface/Subsystem ==
  In1 : Inport
  Demux : Demux  Outputs=3
  Mux : Mux  Inputs=3
  Transfer Fcn : TransferFcn  Denominator=[1e-6 1]
  Transfer Fcn1 : TransferFcn  Denominator=[1e-6 1]
  Transfer Fcn2 : TransferFcn  Denominator=[1e-6 1]
  Out1 : Outport  VectorParamsAs1DForOutWhenUnconnected=off
  wires:
  Demux/2 -> Transfer Fcn2/1
  Demux/1 -> Transfer Fcn/1
  Transfer Fcn1/1 -> Mux/3
  Mux/1 -> Out1/1
  Transfer Fcn2/1 -> Mux/2
  Demux/3 -> Transfer Fcn1/1
  Transfer Fcn/1 -> Mux/1
  In1/1 -> Demux/1

== system My_gfm_battery_sil_2_ConvIGBT_zDomain/ac Network with MVT (native math)4/Network Interface/Subsystem1 ==
  In1 : Inport
  Demux : Demux  Outputs=3
  Mux : Mux  Inputs=3
  Transfer Fcn : TransferFcn  Denominator=[1e-6 1]
  Transfer Fcn1 : TransferFcn  Denominator=[1e-6 1]
  Transfer Fcn2 : TransferFcn  Denominator=[1e-6 1]
  Out1 : Outport  VectorParamsAs1DForOutWhenUnconnected=off
  wires:
  Demux/2 -> Transfer Fcn2/1
  Demux/1 -> Transfer Fcn/1
  Transfer Fcn1/1 -> Mux/3
  Mux/1 -> Out1/1
  Transfer Fcn2/1 -> Mux/2
  Demux/3 -> Transfer Fcn1/1
  Transfer Fcn/1 -> Mux/1
  In1/1 -> Demux/1

== system My_gfm_battery_sil_2_ConvIGBT_zDomain/ac Network with MVT (native math)4/Network Interface/VSI1 ==
  V : Inport
  Controlled Voltage Source : spsControlledVoltageSourceLib/Controlled Voltage Source  Initialize=off  Source_Type=AC  Amplitude=0  Phase=0  Frequency=0  Measurements=None
  Controlled Voltage Source1 : spsControlledVoltageSourceLib/Controlled Voltage Source  Initialize=off  Source_Type=AC  Amplitude=0  Phase=0  Frequency=0  Measurements=None
  Demux : Demux  Outputs=3
  Terminator : Terminator
  A : PMIOPort  Side=Right
  B : PMIOPort  Port=2  Side=Right
  C : PMIOPort  Port=3  Side=Right
  wires:
  Demux/1 -> Controlled Voltage Source/1
  Demux/2 -> Controlled Voltage Source1/1
  V/1 -> Demux/1
  Demux/3 -> Terminator/1
  connections:
  Controlled Voltage Source/RConn1 -- A/RConn1
  Controlled Voltage Source1/RConn1 -- B/RConn1
  Controlled Voltage Source1/LConn1 -- Controlled Voltage Source/LConn1 -- C/RConn1

== system My_gfm_battery_sil_2_ConvIGBT_zDomain/ac Network with MVT (native math)4/Network Interface/Volt Meas1 ==
  Ground : Ground
  Mux : Mux  Inputs=3
  V_AB : spsVoltageMeasurementLib/Voltage Measurement  PhasorSimulation=off  OutputType=Complex  PSBequivalent=0
  V_BC : spsVoltageMeasurementLib/Voltage Measurement  PhasorSimulation=off  OutputType=Complex  PSBequivalent=0
  A : PMIOPort  Side=Left
  B : PMIOPort  Port=2  Side=Left
  C : PMIOPort  Port=3  Side=Left
  V : Outport  VectorParamsAs1DForOutWhenUnconnected=off
  wires:
  V_AB/1 -> Mux/1
  V_BC/1 -> Mux/2
  Mux/1 -> V/1  "[Vab,Vbc]"
  Ground/1 -> Mux/3
  connections:
  V_BC/LConn1 -- B/RConn1
  A/RConn1 -- V_AB/LConn1
  C/RConn1 -- V_AB/LConn2 -- V_BC/LConn2

== system My_gfm_battery_sil_2_ConvIGBT_zDomain/ac Network with MVT (native math)4/Network Interface1/CSI2 ==
  I : Inport
  Demux : Demux  Outputs=3
  Series RLC Branch : spsSeriesRLCBranchLib/Series RLC Branch  LConnTagsString=__new0  RConnTagsString=__new0  BranchType=R  Resistance=1e3  Inductance=1e-3  SetiL0=off  InitialCurrent=0  Capacitance=1e-6  Setx0=off  InitialVoltage=0  Measurements=None
  Series RLC Branch1 : spsSeriesRLCBranchLib/Series RLC Branch  LConnTagsString=__new0  RConnTagsString=__new0  BranchType=R  Resistance=1e3  Inductance=1e-3  SetiL0=off  InitialCurrent=0  Capacitance=1e-6  Setx0=off  InitialVoltage=0  Measurements=None
  Series RLC Branch2 : spsSeriesRLCBranchLib/Series RLC Branch  LConnTagsString=__new0  RConnTagsString=__new0  BranchType=R  Resistance=1e3  Inductance=1e-3  SetiL0=off  InitialCurrent=0  Capacitance=1e-6  Setx0=off  InitialVoltage=0  Measurements=None
  iA : spsControlledCurrentSourceLib/Controlled Current Source  Initialize=off  Source_Type=AC  Amplitude=0  Phase=0  Frequency=0  Measurements=None
  iB : spsControlledCurrentSourceLib/Controlled Current Source  Initialize=off  Source_Type=AC  Amplitude=0  Phase=0  Frequency=0  Measurements=None
  iB1 : spsControlledCurrentSourceLib/Controlled Current Source  Initialize=off  Source_Type=AC  Amplitude=0  Phase=0  Frequency=0  Measurements=None
  A : PMIOPort  Side=Right
  B : PMIOPort  Port=2  Side=Right
  C : PMIOPort  Port=3  Side=Right
  wires:
  Demux/1 -> iA/1
  Demux/2 -> iB/1
  I/1 -> Demux/1
  Demux/3 -> iB1/1
  connections:
  iA/RConn1 -- A/RConn1 -- Series RLC Branch/LConn1
  iB/RConn1 -- B/RConn1 -- Series RLC Branch1/LConn1
  Series RLC Branch1/RConn1 -- Series RLC Branch/RConn1 -- iA/LConn1 -- iB/LConn1 -- iB1/LConn1 -- Series RLC Branch2/RConn1
  C/RConn1 -- iB1/RConn1 -- Series RLC Branch2/LConn1

== system My_gfm_battery_sil_2_ConvIGBT_zDomain/ac Network with MVT (native math)4/Network Interface1/Cur Meas ==
  Current Measurement : spsCurrentMeasurementLib/Current Measurement  PhasorSimulation=off  OutputType=Complex  PSBequivalent=0
  Current Measurement1 : spsCurrentMeasurementLib/Current Measurement  PhasorSimulation=off  OutputType=Complex  PSBequivalent=0
  Current Measurement2 : spsCurrentMeasurementLib/Current Measurement  PhasorSimulation=off  OutputType=Complex  PSBequivalent=0
  Mux : Mux  Inputs=3
  A : PMIOPort  Side=Left
  B : PMIOPort  Port=2  Side=Left
  C : PMIOPort  Port=3  Side=Left
  a : PMIOPort  Port=4  Side=Right
  b : PMIOPort  Port=5  Side=Right
  c : PMIOPort  Port=6  Side=Right
  I : Outport  VectorParamsAs1DForOutWhenUnconnected=off
  wires:
  Current Measurement/1 -> Mux/1
  Current Measurement1/1 -> Mux/2
  Mux/1 -> I/1
  Current Measurement2/1 -> Mux/3
  connections:
  Current Measurement1/LConn1 -- B/RConn1
  Current Measurement/LConn1 -- A/RConn1
  Current Measurement2/LConn1 -- C/RConn1
  a/RConn1 -- Current Measurement/RConn1
  b/RConn1 -- Current Measurement1/RConn1
  c/RConn1 -- Current Measurement2/RConn1

== system My_gfm_battery_sil_2_ConvIGBT_zDomain/ac Network with MVT (native math)4/Network Interface1/Subsystem ==
  In1 : Inport
  Demux : Demux  Outputs=3
  Mux : Mux  Inputs=3
  Transfer Fcn : TransferFcn  Denominator=[1e-6 1]
  Transfer Fcn1 : TransferFcn  Denominator=[1e-6 1]
  Transfer Fcn2 : TransferFcn  Denominator=[1e-6 1]
  Out1 : Outport  VectorParamsAs1DForOutWhenUnconnected=off
  wires:
  Demux/2 -> Transfer Fcn2/1
  Demux/1 -> Transfer Fcn/1
  Transfer Fcn1/1 -> Mux/3
  Mux/1 -> Out1/1
  Transfer Fcn2/1 -> Mux/2
  Demux/3 -> Transfer Fcn1/1
  Transfer Fcn/1 -> Mux/1
  In1/1 -> Demux/1

== system My_gfm_battery_sil_2_ConvIGBT_zDomain/ac Network with MVT (native math)4/Network Interface1/Subsystem1 ==
  In1 : Inport
  Demux : Demux  Outputs=3
  Mux : Mux  Inputs=3
  Transfer Fcn : TransferFcn  Denominator=[1e-6 1]
  Transfer Fcn1 : TransferFcn  Denominator=[1e-6 1]
  Transfer Fcn2 : TransferFcn  Denominator=[1e-6 1]
  Out1 : Outport  VectorParamsAs1DForOutWhenUnconnected=off
  wires:
  Demux/2 -> Transfer Fcn2/1
  Demux/1 -> Transfer Fcn/1
  Transfer Fcn1/1 -> Mux/3
  Mux/1 -> Out1/1
  Transfer Fcn2/1 -> Mux/2
  Demux/3 -> Transfer Fcn1/1
  Transfer Fcn/1 -> Mux/1
  In1/1 -> Demux/1

== system My_gfm_battery_sil_2_ConvIGBT_zDomain/ac Network with MVT (native math)4/Network Interface1/VSI1 ==
  V : Inport
  Controlled Voltage Source : spsControlledVoltageSourceLib/Controlled Voltage Source  Initialize=off  Source_Type=AC  Amplitude=0  Phase=0  Frequency=0  Measurements=None
  Controlled Voltage Source1 : spsControlledVoltageSourceLib/Controlled Voltage Source  Initialize=off  Source_Type=AC  Amplitude=0  Phase=0  Frequency=0  Measurements=None
  Demux : Demux  Outputs=3
  Terminator : Terminator
  A : PMIOPort  Side=Right
  B : PMIOPort  Port=2  Side=Right
  C : PMIOPort  Port=3  Side=Right
  wires:
  Demux/1 -> Controlled Voltage Source/1
  Demux/2 -> Controlled Voltage Source1/1
  V/1 -> Demux/1
  Demux/3 -> Terminator/1
  connections:
  Controlled Voltage Source/RConn1 -- A/RConn1
  Controlled Voltage Source1/RConn1 -- B/RConn1
  Controlled Voltage Source1/LConn1 -- Controlled Voltage Source/LConn1 -- C/RConn1

== system My_gfm_battery_sil_2_ConvIGBT_zDomain/ac Network with MVT (native math)4/Network Interface1/Volt Meas1 ==
  Ground : Ground
  Mux : Mux  Inputs=3
  V_AB : spsVoltageMeasurementLib/Voltage Measurement  PhasorSimulation=off  OutputType=Complex  PSBequivalent=0
  V_BC : spsVoltageMeasurementLib/Voltage Measurement  PhasorSimulation=off  OutputType=Complex  PSBequivalent=0
  A : PMIOPort  Side=Left
  B : PMIOPort  Port=2  Side=Left
  C : PMIOPort  Port=3  Side=Left
  V : Outport  VectorParamsAs1DForOutWhenUnconnected=off
  wires:
  V_AB/1 -> Mux/1
  V_BC/1 -> Mux/2
  Mux/1 -> V/1  "[Vab,Vbc]"
  Ground/1 -> Mux/3
  connections:
  V_BC/LConn1 -- B/RConn1
  A/RConn1 -- V_AB/LConn1
  C/RConn1 -- V_AB/LConn2 -- V_BC/LConn2

== system My_gfm_battery_sil_2_ConvIGBT_zDomain/ac Network with MVT (native math)4/Two-Level Converter1/Model1 ==
  note: (Uref)
  g : Inport  SampleTime=Ts
  Block : Inport  Port=2
  Add : Sum  Inputs=+-
  Constant : Constant
  Constant1 : Constant  Value=0
  Constant2 : Constant
  Current Measurement : spsCurrentMeasurementLib/Current Measurement  PhasorSimulation=off  OutputType=Complex  PSBequivalent=0
  Data Type Conversion2 : DataTypeConversion  OutDataTypeStr=double  SaturateOnIntegerOverflow=off  RndMeth=Floor
  Demux : Demux  Outputs=2
  Fcn2 : Fcn  Expr=(u(1)+1)*0.5
  MATLAB Function : MATLAB Function  TreatAsAtomicUnit=on
  Mux : Mux  Inputs=2
  Mux1 : Mux  Inputs=2
  Power : spsHalfBridgeModel/Power  SystemSampleTime=-1  VariantActivationTime=update diagram  EmptyChoice=off  PassThrough=off  PassThroughVariantControl=(default)  EmptyChoiceVariantControl=(default)  AllowFlexibleInterface=on  Latency=0  AutoFrameSizeCalculation=off
  Product2 : Product
  Product8 : Product
  Saturation : Saturate  UpperLimit=1.0  LowerLimit=-1.0
  Scope : Scope  NumInputPorts=2
      settings: ActiveDisplayYMinimum=-0.125  ActiveDisplayYMaximum=1.125
  Scope1 : Scope  NumInputPorts=2
      settings: ActiveDisplayYMinimum=0.0581  ActiveDisplayYMaximum=0.93277  DataLoggingVariableName=ScopeData2
  Scope2 : Scope  NumInputPorts=6
      settings: ActiveDisplayYMinimum=-1057.03298  ActiveDisplayYMaximum=1237.20421  DataLoggingVariableName=ScopeData3
  Switch : Switch  Criteria=u2 > Threshold  SaturateOnIntegerOverflow=off  InputSameDT=off
  Transfer Fcn : TransferFcn  Denominator=[1e-6 1]
  Transfer Fcn1 : TransferFcn  Denominator=[1e-6 1]
  Transfer Fcn2 : TransferFcn  Denominator=[1e-6 1]
  Voltage Measurement : spsVoltageMeasurementLib/Voltage Measurement  PhasorSimulation=off  OutputType=Complex  PSBequivalent=0
  + : PMIOPort  Tag=PMCPort  Side=Right
  - : PMIOPort  Tag=PMCPort  Port=2  Side=Right
  Out : PMIOPort  Tag=PMCPort  Port=3  Side=Left
  wires:
  Saturation/1 -> Fcn2/1
  g/1 -> Saturation/1
  Block/1 -> Switch/2, Scope/1
  Data Type Conversion2/1 -> Scope/2, Product2/1, Product8/1
  Product2/1 -> Mux1/1
  Product8/1 -> Mux1/2
  Add/1 -> Scope1/2, Product8/2
  Constant/1 -> Add/1
  Fcn2/1 -> Add/2, Scope1/1, Product2/2
  Switch/1 -> Data Type Conversion2/1
  Power/2 -> Scope2/4, Demux/1
  Demux/2 -> Transfer Fcn2/1
  Demux/1 -> Transfer Fcn/1
  Transfer Fcn/1 -> Mux/1
  Transfer Fcn2/1 -> Mux/2
  Mux/1 -> MATLAB Function/3(I)
  Transfer Fcn1/1 -> MATLAB Function/2(Vdc)
  Power/1 -> Scope2/2, Transfer Fcn1/1
  MATLAB Function/2(Idc) -> Power/2, Scope2/3
  MATLAB Function/1(V) -> Power/1, Scope2/1
  Mux1/1 -> MATLAB Function/1(g)
  Constant1/1 -> Switch/1
  Constant2/1 -> Switch/3
  Voltage Measurement/1 -> Scope2/5
  Current Measurement/1 -> Scope2/6
  connections:
  Power/LConn1 -- Current Measurement/LConn1 -- Voltage Measurement/LConn1
  Power/RConn2 -- Voltage Measurement/LConn2 -- -/RConn1
  Power/RConn1 -- +/RConn1
  Current Measurement/RConn1 -- Out/RConn1

== system My_gfm_battery_sil_2_ConvIGBT_zDomain/ac Network with MVT (native math)4/Two-Level Converter1/Model2 ==
  note: (Uref)
  g : Inport  SampleTime=Ts
  Block : Inport  Port=2
  Add : Sum  Inputs=+-
  Constant : Constant
  Constant1 : Constant  Value=0
  Constant2 : Constant
  Data Type Conversion2 : DataTypeConversion  OutDataTypeStr=double  SaturateOnIntegerOverflow=off  RndMeth=Floor
  Demux : Demux  Outputs=2
  Fcn2 : Fcn  Expr=(u(1)+1)*0.5
  MATLAB Function : MATLAB Function  TreatAsAtomicUnit=on
  Mux : Mux  Inputs=2
  Mux1 : Mux  Inputs=2
  Power : spsHalfBridgeModel/Power  SystemSampleTime=-1  VariantActivationTime=update diagram  EmptyChoice=off  PassThrough=off  PassThroughVariantControl=(default)  EmptyChoiceVariantControl=(default)  AllowFlexibleInterface=on  Latency=0  AutoFrameSizeCalculation=off
  Product2 : Product
  Product8 : Product
  Saturation : Saturate  UpperLimit=1.0  LowerLimit=-1.0
  Scope : Scope  NumInputPorts=2
      settings: ActiveDisplayYMinimum=-0.125  ActiveDisplayYMaximum=1.125
  Scope1 : Scope  NumInputPorts=2
      settings: ActiveDisplayYMinimum=-0.0256  ActiveDisplayYMaximum=0.96024  DataLoggingVariableName=ScopeData2
  Scope2 : Scope  NumInputPorts=5
      settings: ActiveDisplayYMinimum=-1250  ActiveDisplayYMaximum=1079.00943  DataLoggingVariableName=ScopeData3
  Switch : Switch  Criteria=u2 > Threshold  SaturateOnIntegerOverflow=off  InputSameDT=off
  Transfer Fcn : TransferFcn  Denominator=[1e-6 1]
  Transfer Fcn1 : TransferFcn  Denominator=[1e-6 1]
  Transfer Fcn2 : TransferFcn  Denominator=[1e-6 1]
  Voltage Measurement : spsVoltageMeasurementLib/Voltage Measurement  PhasorSimulation=off  OutputType=Complex  PSBequivalent=0
  + : PMIOPort  Tag=PMCPort  Side=Right
  - : PMIOPort  Tag=PMCPort  Port=2  Side=Right
  Out : PMIOPort  Tag=PMCPort  Port=3  Side=Left
  wires:
  Saturation/1 -> Fcn2/1
  g/1 -> Saturation/1
  Block/1 -> Switch/2, Scope/1
  Data Type Conversion2/1 -> Scope/2, Product2/1, Product8/1
  Product2/1 -> Mux1/1
  Product8/1 -> Mux1/2
  Add/1 -> Scope1/2, Product8/2
  Constant/1 -> Add/1
  Fcn2/1 -> Add/2, Scope1/1, Product2/2
  Switch/1 -> Data Type Conversion2/1
  Power/2 -> Scope2/4, Demux/1
  Demux/2 -> Transfer Fcn2/1
  Demux/1 -> Transfer Fcn/1
  Transfer Fcn/1 -> Mux/1
  Transfer Fcn2/1 -> Mux/2
  Mux/1 -> MATLAB Function/3(I)
  Transfer Fcn1/1 -> MATLAB Function/2(Vdc)
  Power/1 -> Scope2/2, Transfer Fcn1/1
  MATLAB Function/2(Idc) -> Power/2, Scope2/3
  MATLAB Function/1(V) -> Power/1, Scope2/1
  Mux1/1 -> MATLAB Function/1(g)
  Constant1/1 -> Switch/1
  Constant2/1 -> Switch/3
  Voltage Measurement/1 -> Scope2/5
  connections:
  Out/RConn1 -- Power/LConn1 -- Voltage Measurement/LConn1
  -/RConn1 -- Power/RConn2 -- Voltage Measurement/LConn2
  Power/RConn1 -- +/RConn1
